simulink model "Smart_DC_Fast_Charging"  (R2026a)
settings: Solver=ode14x  StopTime=7200  FixedStep=1
values from neighbouring files (symbols this model uses):
  var_C_Max = 0.9    [matlab.mat]    (also in predictive_cloud_manager.m = 1.5)
  var_Q = 50 * var_SOH    (= 50)    [generate_thermal_data.m]    (also in matlab.mat = 39; predictive_cloud_manager.m = 39; run_accelerated_aging.m)
  var_R = 0.050 * (1 + 2 * (1 - var_SOH))    (= 0.05)    [generate_thermal_data.m]    (also in matlab.mat = 0.072; predictive_cloud_manager.m = 0.072; run_accelerated_aging.m)
  var_SOH = var_SOH - degradation    [generate_thermal_data.m]    (also in matlab.mat = 0.78; predictive_cloud_manager.m = 0.78; run_accelerated_aging.m = var_SOH - total_degradation)
libraries: fl_lib x9, nesl_utility x5, batteryecm_lib x1
settings Model: Creator=thanu  LastModifiedBy=thanu

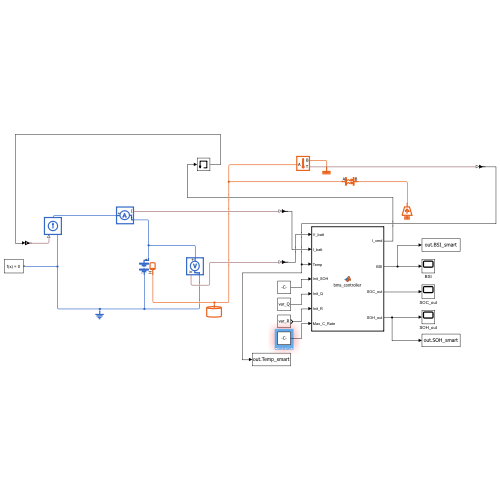
[thumbnail: Simulink's stored preview of the top-level diagram]
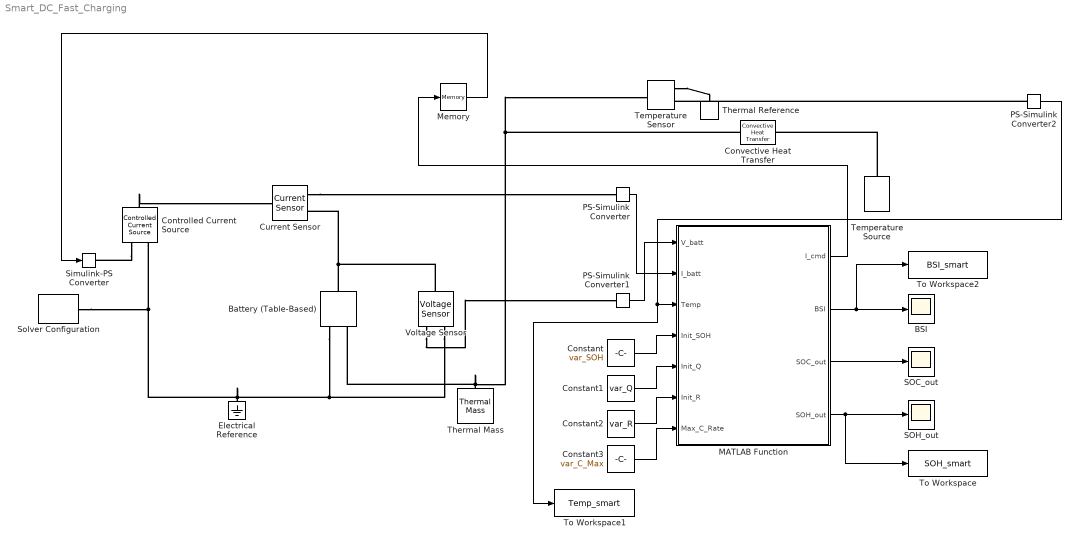
== system Smart_DC_Fast_Charging ==
  BSI : Scope
      settings: ActiveDisplayYMinimum=0  ActiveDisplayYMaximum=60  DataLoggingMaxPoints=7200
  Battery (Table-Based) : batteryecm_lib/Battery (Table-Based)  SOC_vec=[0, 0.1, 0.2, 0.3, 0.4, 0.5, 0.6, 0.7, 0.8, 0.9, 1]  T_dependence=simscape.enum.tablebattery.temperature_dependence.no  prm_dir=simscape.enum.tablebattery.prm_dir.noCurrentDirectionality  T_vec=[278, 293, 313] K  V0_mat=[3.49, 3.5, 3.51; 3.55, 3.57, 3.56; 3.62, 3.63, 3.64; 3.71, 3.71, 3.72; 3.91, 3.93, 3.94; 4.07, 4.08, 4.08; 4.19, 4.19, 4.19] V  V0_vec=[40, 41.2, 42.8, 44.2, 45.3, 46.2, 47.1, 48, 50.2, 52.8, 54.6] V  V_range=[0, inf] V  R0_mat=[.0117, .0085, .009; .011, .0085, .009; .0114, .0087, .0092; .0107, .0082, .0088; .0107, .0083, .0091; .0113, .0085, .0089; .0116, .0085, .0089] Ohm  R0_vec=[0.05, 0.05, 0.05, 0.05, 0.05, 0.05, 0.05, 0.05, 0.05, 0.05, 0.05] Ohm  R0_dis_mat=[.0117, .0085, .009; .011, .0085, .009; .0114, .0087, .0092; .0107, .0082, .0088; .0107, .0083, .0091; .0113, .0085, .0089; .0116, .0085, .0089] Ohm  R0_dis_vec=[.0085, .0085, .0087, .0082, .0083, .0085, .0085] Ohm  R0_ch_mat=[.0117, .0085, .009; .011, .0085, .009; .0114, .0087, .0092; .0107, .0082, .0088; .0107, .0083, .0091; .0113, .0085, .0089; .0116, .0085, .0089] Ohm  R0_ch_vec=[.0085, .0085, .0087, .0082, .0083, .0085, .0085] Ohm  AH=50 A*hr  prm_leak=simscape.enum.tablebattery.prm_leak.disabled  Rleak_vec=[8000, 7000, 6000] Ohm  Rleak=7e3 Ohm  extrapolation_option=simscape.enum.extrapolation.nearest  SOC_port=simscape.enum.tablebattery.enable.no  prm_dyn=simscape.enum.tablebattery.prm_dyn.off  R1_mat=[.0109, .0029, .0013; .0069, .0024, .0012; .0047, .0026, .0013; .0034, .0016, .001; .0033, .0023, .0014; .0033, .0018, .0011; .0028, .0017, .0011] Ohm  R1_vec=[.0029, .0024, .0026, .0016, .0023, .0018, .0017] Ohm  tau1_mat=[20, 36, 39; 31, 45, 39; 109, 105, 61; 36, 29, 26; 59, 77, 67; 40, 33, 29; 25, 39, 33] s  tau1_vec=[36, 45, 105, 29, 77, 33, 39] s  R2_mat=[.0109, .0029, .0013; .0069, .0024, .0012; .0047, .0026, .0013; .0034, .0016, .001; .0033, .0023, .0014; .0033, .0018, .0011; .0028, .0017, .0011] Ohm  R2_vec=[.0029, .0024, .0026, .0016, .0023, .0018, .0017] Ohm  tau2_mat=[20, 36, 39; 31, 45, 39; 109, 105, 61; 36, 29, 26; 59, 77, 67; 40, 33, 29; 25, 39, 33] s  tau2_vec=[36, 45, 105, 29, 77, 33, 39] s  R3_mat=[.0109, .0029, .0013; .0069, .0024, .0012; .0047, .0026, .0013; .0034, .0016, .001; .0033, .0023, .0014; .0033, .0018, .0011; .0028, .0017, .0011] Ohm  R3_vec=[.0029, .0024, .0026, .0016, .0023, .0018, .0017] Ohm  tau3_mat=[20, 36, 39; 31, 45, 39; 109, 105, 61; 36, 29, 26; 59, 77, 67; 40, 33, 29; 25, 39, 33] s  tau3_vec=[36, 45, 105, 29, 77, 33, 39] s  R4_mat=[.0109, .0029, .0013; .0069, .0024, .0012; .0047, .0026, .0013; .0034, .0016, .001; .0033, .0023, .0014; .0033, .0018, .0011; .0028, .0017, .0011] Ohm  R4_vec=[.0029, .0024, .0026, .0016, .0023, .0018, .0017] Ohm  tau4_mat=[20, 36, 39; 31, 45, 39; 109, 105, 61; 36, 29, 26; 59, 77, 67; 40, 33, 29; 25, 39, 33] s  tau4_vec=[36, 45, 105, 29, 77, 33, 39] s  R5_mat=[.0109, .0029, .0013; .0069, .0024, .0012; .0047, .0026, .0013; .0034, .0016, .001; .0033, .0023, .0014; .0033, .0018, .0011; .0028, .0017, .0011] Ohm  R5_vec=[.0029, .0024, .0026, .0016, .0023, .0018, .0017] Ohm  tau5_mat=[20, 36, 39; 31, 45, 39; 109, 105, 61; 36, 29, 26; 59, 77, 67; 40, 33, 29; 25, 39, 33] s  tau5_vec=[36, 45, 105, 29, 77, 33, 39] s  prm_fade=simscape.enum.tablebattery.prm_fade.disabled  N0=100  dV0=0  dR0=0  dAH=0  dRleak=0  dR1=0  dR2=0  dR3=0  dR4=0  dR5=0  N0vec=[0, 100, 200, 300]  Tfadevec=[298.15, 323.15] K  dV0vec=[0, 0, 0, 0]  dR0vec=[0, 0, 0, 0]  dAHvec=[0, 0, 0, 0]  dRleakvec=[0, 0, 0, 0]  dR1vec=[0, 0, 0, 0]  dR2vec=[0, 0, 0, 0]  dR3vec=[0, 0, 0, 0]  dR4vec=[0, 0, 0, 0]  dR5vec=[0, 0, 0, 0]  dV0mat=[0, 0; 0, 0; 0, 0; 0, 0]  dR0mat=[0, 0; 0, 0; 0, 0; 0, 0]  dAHmat=[0, 0; 0, 0; 0, 0; 0, 0]  dRleakmat=[0, 0; 0, 0; 0, 0; 0, 0]  dR1mat=[0, 0; 0, 0; 0, 0; 0, 0]  dR2mat=[0, 0; 0, 0; 0, 0; 0, 0]  dR3mat=[0, 0; 0, 0; 0, 0; 0, 0]  dR4mat=[0, 0; 0, 0; 0, 0; 0, 0]  dR5mat=[0, 0; 0, 0; 0, 0; 0, 0]  prm_age_modeling=simscape.enum.tablebattery.prm_age_modeling.equation  storage_dt_age_vec=[0] d  storage_T_age_vec=[273] K  prm_age_OCV=simscape.enum.tablebattery.prm_age_OCV.OCV  OCV_age=0.9  SOC_age=0.6  prm_age_resistance=simscape.enum.tablebattery.prm_age.disabled  OCV_scaling_age_resistance=2.2134e6  OCV_offset_age_resistance=1.632e6  temp_exp_age_resistance=0.515833569 V  t_exp_age_resistance=0.75  T_age_vec_resistance=[273.15, 298.15, 323.15] K  dt_age_vec_resistance=[0, 90, 180, 270] d  dR0_age_vec=[0, 0, 0]  t_meas_dR0_age=100 d  dR0_age_mat=[0, 0, 0; 0, 0, 0; 0, 0, 0; 0, 0, 0]  prm_age_capacity=simscape.enum.tablebattery.prm_age.disabled  OCV_scaling_age_capacity=1.5097e07  OCV_offset_age_capacity=8.3625e06  temp_exp_age_capacity=0.6011 V  t_exp_age_capacity=0.75  T_age_vec_capacity=[273.15, 298.15, 323.15] K  dt_age_vec_capacity=[0, 90, 180, 270] d  dAH_age_vec=[0, 0, 0]  t_meas_dAH_age=100 d  dAH_age_mat=[0, 0, 0; 0, 0, 0; 0, 0, 0; 0, 0, 0]  thermal_port=simscape.enum.thermaleffects.model  temperature=298.15 K  thermal_mass=100 J/K  i_specify=off  i_priority=None  i=0 A  i_nominal_specify=off  i_nominal_value=1  i_nominal_unit=A  v_specify=off  v_priority=None  v=0 V  v_nominal_specify=off  v_nominal_value=1  v_nominal_unit=V  stateOfCharge_specify=on  stateOfCharge_priority=High  stateOfCharge=0.2  stateOfCharge_nominal_specify=off  stateOfCharge_nominal_value=1  stateOfCharge_nominal_unit=1  num_cycles_specify=off  num_cycles_priority=High  num_cycles=0  num_cycles_nominal_specify=off  num_cycles_nominal_value=1  num_cycles_nominal_unit=1  cell_temperature_specify=off  cell_temperature_priority=High  cell_temperature=298.15 K  cell_temperature_nominal_specify=off  cell_temperature_nominal_value=1  cell_temperature_nominal_unit=K
  Constant : Constant  Value=var_SOH
  Constant1 : Constant  Value=var_Q
  Constant2 : Constant  Value=var_R
  Constant3 : Constant  Value=var_C_Max
  Controlled Current Source : fl_lib/Electrical/Electrical Sources/Controlled Current Source
  Convective Heat Transfer : fl_lib/Thermal/Thermal Elements/Convective Heat Transfer  thermal_type=foundation.enum.constant_variable.constant  area=1e-4 m^2  heat_tr_coeff=20 W/(K*m^2)  min_heat_tr_coeff=1e-3 W/(K*m^2)  T_specify=off  T_priority=None  T=0 K  T_nominal_specify=off  T_nominal_value=1  T_nominal_unit=K  Q_specify=off  Q_priority=None  Q=0 W  Q_nominal_specify=off  Q_nominal_value=1  Q_nominal_unit=W
  Current Sensor : fl_lib/Electrical/Electrical Sensors/Current Sensor
  Electrical Reference : fl_lib/Electrical/Electrical Elements/Electrical Reference
  MATLAB Function : MATLAB Function  TreatAsAtomicUnit=on  SystemSampleTime=1
  Memory : Memory
  PS-Simulink Converter : nesl_utility/PS-Simulink Converter  PhysicalDomain=network_engine_domain  SubClassName=ps_output  LeftPortType=input  RightPortType=output  PseudoPeriodic=off  Frequencies=[]  VectorFormat=inherit  Unit=inherit  AffineConversion=off
  PS-Simulink Converter1 : nesl_utility/PS-Simulink Converter  PhysicalDomain=network_engine_domain  SubClassName=ps_output  LeftPortType=input  RightPortType=output  PseudoPeriodic=off  Frequencies=[]  VectorFormat=inherit  Unit=inherit  AffineConversion=off
  PS-Simulink Converter2 : nesl_utility/PS-Simulink Converter  PhysicalDomain=network_engine_domain  SubClassName=ps_output  LeftPortType=input  RightPortType=output  PseudoPeriodic=off  Frequencies=[]  VectorFormat=inherit  Unit=degC  AffineConversion=on
  SOC_out : Scope
      settings: ActiveDisplayYMinimum=-0.2  ActiveDisplayYMaximum=1.05  DataLoggingMaxPoints=7200
  SOH_out : Scope
      settings: ActiveDisplayYMinimum=0.94974732765815384  ActiveDisplayYMaximum=0.950028030149094  DataLoggingMaxPoints=7200  DataLoggingVariableName=ScopeData2
  Simulink-PS Converter : nesl_utility/Simulink-PS Converter  PhysicalDomain=network_engine_domain  SubClassName=ps_input  LeftPortType=input  RightPortType=output  PseudoPeriodic=off  Frequencies=[]  NoiseDistribution=none  NoiseParameters=[]  Unit=A  AffineConversion=off  FilteringAndDerivatives=provide  SimscapeFilterOrder=1  InputFilterTimeConstant=0.001  UdotUserProvided=0
  Solver Configuration : nesl_utility/Solver Configuration  PhysicalDomain=network_engine_domain  SubClassName=solver  LeftPortType=input  RightPortType=generic  Tones=[]  Harmonics=[]  SimulateNoise=off  Profile=off  UseLocalSampling=off  EnableSwitchedLinearOptims=on  FrequencyDomain=off  UseCCode=off  RelTol=0.001  AbsTol=0.001  MinStep=1e-09  ToWorkspace=off  RevertToSquareIcSolve=off  NumHomotopyIterations=100  PhasorMode=off  PhasorModeNumHarmonics=1  ConsistencySolver=NEWTON_XTOL_AFTER_FTOL  CanonicalOrdering=CANONICAL  OptimizeIntermediates=OPTIMIZED  IndexReductionMethod=DerivativeReplacement  DoDC=off  ResidualTolerance=1e-09  ConsistencyTolSource=GLOBAL  ConsistencyAbsTol=0.001  ConsistencyRelTol=0.001  ConsistencyTolFactor=0.001  UseLocalSolver=off  LocalSolverChoice=NE_BACKWARD_EULER_ADVANCER  ResolveIndetEquations=on  FunctionEvalNumThread=1  LocalSolverSampleTime=0.001  DoFixedCost=off  MaxNonlinIter=3  MaxModeIter=2  ComputeImpulses=off  ImpulseIterations=2  LinearAlgebra=auto  LinearAlgebraNumThread=0  EquationFormulation=NE_TIME_EF  DelaysMemoryBudget=1024  AutomaticFiltering=on  FilteringTimeConstant=0.001  PartitionStorageMethod=AS_NEEDED  PartitionMemoryBudget=1024  PartitionMethod=ROBUST  MultibodyUseLocalSolver=off  MultibodyLocalSolverChoice=ODE1  MultibodyLocalSolverSampleTime=0.001
  Temperature Sensor : fl_lib/Thermal/Thermal Sensors/Temperature Sensor  temperature_measure=foundation.enum.MeasurementReference.difference
  Temperature Source : fl_lib/Thermal/Thermal Sources/Temperature Source  temperature=25 degC
  Thermal Mass : fl_lib/Thermal/Thermal Elements/Thermal Mass  mass_type=foundation.enum.constant_variable.constant  mass=50 kg  sp_heat=800 J/(K*kg)  mass_min=1e-6 kg  num_ports=foundation.enum.numPorts2.one  m_specify=off  m_priority=High  m=1 kg  m_nominal_specify=off  m_nominal_value=1  m_nominal_unit=kg  T_specify=on  T_priority=High  T=25 degC  T_nominal_specify=off  T_nominal_value=1  T_nominal_unit=K  Q_specify=off  Q_priority=None  Q=0 W  Q_nominal_specify=off  Q_nominal_value=1  Q_nominal_unit=W
  Thermal Reference : fl_lib/Thermal/Thermal Elements/Thermal Reference
  To Workspace : ToWorkspace  VariableName=SOH_smart  SaveFormat=Timeseries  SampleTime=-1
  To Workspace1 : ToWorkspace  VariableName=Temp_smart  SaveFormat=Timeseries  SampleTime=-1
  To Workspace2 : ToWorkspace  VariableName=BSI_smart  SaveFormat=Timeseries  SampleTime=-1
  Voltage Sensor : fl_lib/Electrical/Electrical Sensors/Voltage Sensor
  wires:
  MATLAB Function/3(SOC_out) -> SOC_out/1
  MATLAB Function/4(SOH_out) -> SOH_out/1, To Workspace/1
  PS-Simulink Converter1/1 -> MATLAB Function/1(V_batt)
  PS-Simulink Converter/1 -> MATLAB Function/2(I_batt)
  MATLAB Function/1(I_cmd) -> Memory/1
  Memory/1 -> Simulink-PS Converter/1
  PS-Simulink Converter2/1 -> To Workspace1/1, MATLAB Function/3(Temp)
  MATLAB Function/2(BSI) -> To Workspace2/1, BSI/1
  Constant/1 -> MATLAB Function/4(Init_SOH)
  Constant1/1 -> MATLAB Function/5(Init_Q)
  Constant2/1 -> MATLAB Function/6(Init_R)
  Constant3/1 -> MATLAB Function/7(Max_C_Rate)
  connections:
  Controlled Current Source/LConn1 -- Current Sensor/LConn1
  Voltage Sensor/LConn1 -- Battery (Table-Based)/LConn1 -- Current Sensor/RConn2
  Battery (Table-Based)/RConn1 -- Voltage Sensor/RConn2 -- Solver Configuration/RConn1 -- Controlled Current Source/RConn2 -- Electrical Reference/LConn1
  Current Sensor/RConn1 -- PS-Simulink Converter/LConn1
  Controlled Current Source/RConn1 -- Simulink-PS Converter/RConn1
  Voltage Sensor/RConn1 -- PS-Simulink Converter1/LConn1
  Convective Heat Transfer/LConn1 -- Battery (Table-Based)/RConn2 -- Thermal Mass/LConn1 -- Temperature Sensor/LConn1
  Temperature Sensor/RConn1 -- Thermal Reference/LConn1
  Temperature Source/LConn1 -- Convective Heat Transfer/RConn1
  PS-Simulink Converter2/LConn1 -- Temperature Sensor/RConn2

== matlab function Smart_DC_Fast_Charging/MATLAB Function ==
  data: V_batt input; I_cmd output; I_batt input; Temp input; BSI output; SOC_out output; SOH_out output; Init_SOH input; Init_Q input; Init_R input; Max_C_Rate input
function [I_cmd, BSI, SOC_out, SOH_out] = bms_controller(V_batt, I_batt, Temp, Init_SOH, Init_Q, Init_R, Max_C_Rate)% Inputs: Measured Voltage, Current, Temp, and Starting Battery Conditions
% Outputs: Current Command, BSI, SOC, SOH
    
    %% 1. Initialize persistent memory (Microcontroller state)
    persistent SOC SOH safety_lockout I_prev
    if isempty(SOC)
        SOC = 0.20; 
        SOH = Init_SOH; % <--- Now accepts aging data from the script
        safety_lockout = false; 
        I_prev = 0; 
    end
    
    %% 2. BMS Parameters
    Q_nom = Init_Q; % <--- Now accepts shrinking capacity
    R_initial = Init_R; % <--- Now accepts growing resistance
    
    V_max = 54.6;
    T_warning = 40; T_max = 45;
    BSI_warning = 45; BSI_high = 60; BSI_trip = 80;
    C_rate_max = Max_C_Rate;
    dt = 1; 
    
    ramp_up_limit = 5; 
    ramp_down_limit = 20; 
    
    %% 3. SOC Coulomb Counting & SOH Degradation
    SOC = SOC + (I_batt * dt) / (Q_nom * 3600);
    SOC = min(max(SOC, 0), 1);
    
    temp_factor = 1 + 0.05 * max(Temp - 25, 0);
    c_rate_factor = 1 + 0.5 * ((I_batt/Q_nom)^2);
    SOH = SOH - (2e-8 * c_rate_factor * temp_factor * dt);
    SOH = min(max(SOH, 0), 1);
    
    %% 4. Internal Resistance Estimation
    soc_norm = abs(SOC - 0.5) / 0.5;
    Rint = R_initial * (1 + 0.30*(soc_norm^1.2)) * (1 + 1.2*max(0,1-SOH)) * min(max(exp(-0.015*(Temp-25)),0.75),1.25);
    
    %% 5. BSI Calculation
    stress_C = min((I_batt/Q_nom)/C_rate_max, 1);
    stress_T = min(max((Temp-25)/(T_max-25), 0), 1);
    if SOC < 0.50; stress_SOC = 0.10;
    elseif SOC < 0.70; stress_SOC = 0.30;
    elseif SOC < 0.85; stress_SOC = 0.55;
    elseif SOC < 0.95; stress_SOC = 0.85;
    else; stress_SOC = 1.00; end
    stress_R = min(max((Rint/R_initial - 1)/0.50, 0), 1);
    stress_SOH = min(max((1-SOH)/0.30, 0), 1);
    
    BSI = 100 * (0.35*stress_C + 0.25*stress_T + 0.20*stress_SOC + 0.10*stress_R + 0.10*stress_SOH);
    BSI = min(max(BSI, 0), 100);
    
    %% 6. Adaptive C-Rate Derating
    if SOC < 0.50; base_C = Max_C_Rate;
    elseif SOC < 0.70; base_C = Max_C_Rate * 0.8;
    elseif SOC < 0.85; base_C = Max_C_Rate * 0.6;
    elseif SOC < 0.90; base_C = Max_C_Rate * 0.45;
    else; base_C = Max_C_Rate * 0.4; end
    
    if Temp < 28; fT = 1.0;
    elseif Temp < 30; fT = 0.90;
    elseif Temp < 32; fT = 0.75;
    elseif Temp < 35; fT = 0.55;
    elseif Temp < T_warning; fT = 0.35;
    else; fT = 0.20; end
    
    if BSI < 35; fB = 1.0;
    elseif BSI < BSI_warning; fB = 0.90;
    elseif BSI < BSI_high; fB = 0.75;
    elseif BSI < BSI_trip; fB = 0.50;
    else; fB = 0; end
    
    C_target = min([base_C, base_C*fT, base_C*fB, C_rate_max]);
    I_CC = C_target * Q_nom;
    
    %% 7. Constant Voltage (CV) Limitation
    OCV_est = V_batt - (I_batt * Rint);
    I_CV = max((V_max - OCV_est) / Rint, 0);
    I_target = min(I_CC, I_CV);
    
    %% 8. Software Slew Rate Limiter
    if I_target > I_prev
        I_cmd = min(I_target, I_prev + ramp_up_limit * dt);
    elseif I_target < I_prev
        I_cmd = max(I_target, I_prev - ramp_down_limit * dt);
    else
        I_cmd = I_target;
    end
    
    %% 9. HYSTERESIS SAFETY LOCKOUT
    if V_batt > V_max + 0.05 || Temp >= T_max || BSI >= BSI_trip || SOC >= 0.95
        safety_lockout = true;
    end
    if safety_lockout == true
        if Temp < (T_max - 3) && BSI < (BSI_trip - 10) && V_batt <= V_max && SOC < 0.95
            safety_lockout = false;
        end
    end
    if safety_lockout == true
        I_cmd = 0;
    end
    I_prev = I_cmd;
    
    %% 10. Outputs
    SOC_out = SOC;
    SOH_out = SOH;
end
